simulink model "rfdc"  (R2021a)
(part 2 of 3)

      mask DialogControl t226_ADCPair23 Prompt: ADC Pair 2,3
      mask DialogControl t226_QT_adc2 Prompt: ADC 2
      mask DialogControl t226_QT_adc2_DataSettings Prompt: Data Settings
      mask DialogControl t226_QT_adc2_req_axis_clk_label Prompt: Required AXI4-Stream clock:
      mask DialogControl t226_QT_adc2_MixerSettings Prompt: MIxer Settings
      mask DialogControl t226_QT_adc2_AnalogSettings Prompt: Analog Settings
      mask DialogControl t226_QT_adc3 Prompt: ADC 3
      mask DialogControl t226_QT_adc3_DataSettings Prompt: Data Settings
      mask DialogControl t226_QT_adc3_req_axis_clk_label Prompt: Required AXI4-Stream clock:
      mask DialogControl t226_QT_adc3_MixerSettings Prompt: MIxer Settings
      mask DialogControl t226_QT_adc3_AnalogSettings Prompt: Analog Settings
      mask DialogControl t226_DualTileConfig Prompt: Dual Tile Configuration
      mask DialogControl t226_DT_adc0 Prompt: ADC 0
      mask DialogControl t226_DT_adc0_DataSettings Prompt: Data Settings
      mask DialogControl t226_DT_adc0_req_axis_clk_label Prompt: Required AXI4-Stream clock:
      mask DialogControl t226_DT_adc0_MixerSettings Prompt: MIxer Settings
      mask DialogControl t226_DT_adc0_AnalogSettings Prompt: Analog Settings
      mask DialogControl t226_DT_adc1 Prompt: ADC 1
      mask DialogControl t226_DT_adc1_DataSettings Prompt: Data Settings
      mask DialogControl t226_DT_adc1_req_axis_clk_label Prompt: Required AXI4-Stream clock:
      mask DialogControl t226_DT_adc1_MixerSettings Prompt: MIxer Settings
      mask DialogControl t226_DT_adc1_AnalogSettings Prompt: Analog Settings
      mask DialogControl Tile227_container Prompt: Tile 227
      mask DialogControl pll_clocking_config_227 Prompt: Clocking and PLL Configuration
      mask DialogControl t227_QuadTileConfig Prompt: Quad Tile Configuration
      mask DialogControl t227_ADCPair01 Prompt: ADC Pair 0,1
      mask DialogControl t227_QT_adc0 Prompt: ADC 0
      mask DialogControl t227_QT_adc0_DataSettings Prompt: Data Settings
      mask DialogControl t227_QT_adc0_req_axis_clk_label Prompt: Required AXI4-Stream clock:
      mask DialogControl t227_QT_adc0_MixerSettings Prompt: MIxer Settings
      mask DialogControl t227_QT_adc0_AnalogSettings Prompt: Analog Settings
      mask DialogControl t227_QT_adc1 Prompt: ADC 1
      mask DialogControl t227_QT_adc1_DataSettings Prompt: Data Settings
      mask DialogControl t227_QT_adc1_req_axis_clk_label Prompt: Required AXI4-Stream clock:
      mask DialogControl t227_QT_adc1_MixerSettings Prompt: MIxer Settings
      mask DialogControl t227_QT_adc1_AnalogSettings Prompt: Analog Settings
      mask DialogControl t227_ADCPair23 Prompt: ADC Pair 2,3
      mask DialogControl t227_QT_adc2 Prompt: ADC 2
      mask DialogControl t227_QT_adc2_DataSettings Prompt: Data Settings
      mask DialogControl t227_QT_adc2_req_axis_clk_label Prompt: Required AXI4-Stream clock:
      mask DialogControl t227_QT_adc2_MixerSettings Prompt: MIxer Settings
      mask DialogControl t227_QT_adc2_AnalogSettings Prompt: Analog Settings
      mask DialogControl t227_QT_adc3 Prompt: ADC 3
      mask DialogControl t227_QT_adc3_DataSettings Prompt: Data Settings
      mask DialogControl t227_QT_adc3_req_axis_clk_label Prompt: Required AXI4-Stream clock:
      mask DialogControl t227_QT_adc3_MixerSettings Prompt: MIxer Settings
      mask DialogControl t227_QT_adc3_AnalogSettings Prompt: Analog Settings
      mask DialogControl t227_DualTileConfig Prompt: Dual Tile Configuration
      mask DialogControl t227_DT_adc0 Prompt: ADC 0
      mask DialogControl t227_DT_adc0_DataSettings Prompt: Data Settings
      mask DialogControl t227_DT_adc0_req_axis_clk_label Prompt: Required AXI4-Stream clock:
      mask DialogControl t227_DT_adc0_MixerSettings Prompt: MIxer Settings
      mask DialogControl t227_DT_adc0_AnalogSettings Prompt: Analog Settings
      mask DialogControl t227_DT_adc1 Prompt: ADC 1
      mask DialogControl t227_DT_adc1_DataSettings Prompt: Data Settings
      mask DialogControl t227_DT_adc1_req_axis_clk_label Prompt: Required AXI4-Stream clock:
      mask DialogControl t227_DT_adc1_MixerSettings Prompt: MIxer Settings
      mask DialogControl t227_DT_adc1_AnalogSettings Prompt: Analog Settings
      mask DialogControl DACTileSelect Prompt: DAC Tiles
      mask DialogControl Tile228_container Prompt: Tile 228
      mask DialogControl pll_clocking_config_228 Prompt: Clocking and PLL Configuration
      mask DialogControl t228_QuadTileConfig Prompt: Quad Tile Configuration
      mask DialogControl t228_DACPair01 Prompt: DAC Pair 0,1
      mask DialogControl t228_QT_dac0 Prompt: DAC 0
      mask DialogControl t228_QT_dac0_DataSettings Prompt: Data Settings
      mask DialogControl t228_QT_dac0_req_axis_clk_label Prompt: Required AXI4-Stream clock:
      mask DialogControl t228_QT_dac0_MixerSettings Prompt: MIxer Settings
      mask DialogControl t228_QT_dac0_AnalogSettings Prompt: Analog Settings
      mask DialogControl t228_QT_dac1 Prompt: DAC 1
      mask DialogControl t228_QT_dac1_DataSettings Prompt: Data Settings
      mask DialogControl t228_QT_dac1_req_axis_clk_label Prompt: Required AXI4-Stream clock:
      mask DialogControl t228_QT_dac1_MixerSettings Prompt: MIxer Settings
      mask DialogControl t228_QT_dac1_AnalogSettings Prompt: Analog Settings
      mask DialogControl t228_DACPair23 Prompt: DAC Pair 2,3
      mask DialogControl t228_QT_dac2 Prompt: DAC 2
      mask DialogControl t228_QT_dac2_DataSettings Prompt: Data Settings
      mask DialogControl t228_QT_dac2_req_axis_clk_label Prompt: Required AXI4-Stream clock:
      mask DialogControl t228_QT_dac2_MixerSettings Prompt: MIxer Settings
      mask DialogControl t228_QT_dac2_AnalogSettings Prompt: Analog Settings
      mask DialogControl t228_QT_dac3 Prompt: DAC 3
      mask DialogControl t228_QT_dac3_DataSettings Prompt: Data Settings
      mask DialogControl t228_QT_dac3_req_axis_clk_label Prompt: Required AXI4-Stream clock:
      mask DialogControl t228_QT_dac3_MixerSettings Prompt: MIxer Settings
      mask DialogControl t228_QT_dac3_AnalogSettings Prompt: Analog Settings
      mask DialogControl t228_DualTileConfig Prompt: Dual Tile Configuration
      mask DialogControl t228_DT_dac0 Prompt: DAC 0
      mask DialogControl t228_DT_dac0_DataSettings Prompt: Data Settings
      mask DialogControl t228_DT_dac0_req_axis_clk_label Prompt: Required AXI4-Stream clock:
      mask DialogControl t228_DT_dac0_MixerSettings Prompt: MIxer Settings
      mask DialogControl t228_DT_dac0_AnalogSettings Prompt: Analog Settings
      mask DialogControl t228_DT_dac1 Prompt: DAC 1
      mask DialogControl t228_DT_dac1_DataSettings Prompt: Data Settings
      mask DialogControl t228_DT_dac1_req_axis_clk_label Prompt: Required AXI4-Stream clock:
      mask DialogControl t228_DT_dac1_MixerSettings Prompt: MIxer Settings
      mask DialogControl t228_DT_dac1_AnalogSettings Prompt: Analog Settings
      mask DialogControl Tile229_container Prompt: Tile 229
      mask DialogControl pll_clocking_config_229 Prompt: Clocking and PLL Configuration
      mask DialogControl t229_QuadTileConfig Prompt: Quad Tile Configuration
      mask DialogControl t229_DACPair01 Prompt: DAC Pair 0,1
      mask DialogControl t229_QT_dac0 Prompt: DAC 0
      mask DialogControl t229_QT_dac0_DataSettings Prompt: Data Settings
      mask DialogControl t229_QT_dac0_req_axis_clk_label Prompt: Required AXI4-Stream clock:
      mask DialogControl t229_QT_dac0_MixerSettings Prompt: MIxer Settings
      mask DialogControl t229_QT_dac0_AnalogSettings Prompt: Analog Settings
      mask DialogControl t229_QT_dac1 Prompt: DAC 1
      mask DialogControl t229_QT_dac1_DataSettings Prompt: Data Settings
      mask DialogControl t229_QT_dac1_req_axis_clk_label Prompt: Required AXI4-Stream clock:
      mask DialogControl t229_QT_dac1_MixerSettings Prompt: MIxer Settings
      mask DialogControl t229_QT_dac1_AnalogSettings Prompt: Analog Settings
      mask DialogControl t229_DACPair23 Prompt: DAC Pair 2,3
      mask DialogControl t229_QT_dac2 Prompt: DAC 2
      mask DialogControl t229_QT_dac2_DataSettings Prompt: Data Settings
      mask DialogControl t229_QT_dac2_req_axis_clk_label Prompt: Required AXI4-Stream clock:
      mask DialogControl t229_QT_dac2_MixerSettings Prompt: MIxer Settings
      mask DialogControl t229_QT_dac2_AnalogSettings Prompt: Analog Settings
      mask DialogControl t229_QT_dac3 Prompt: DAC 3
      mask DialogControl t229_QT_dac3_DataSettings Prompt: Data Settings
      mask DialogControl t229_QT_dac3_req_axis_clk_label Prompt: Required AXI4-Stream clock:
      mask DialogControl t229_QT_dac3_MixerSettings Prompt: MIxer Settings
      mask DialogControl t229_QT_dac3_AnalogSettings Prompt: Analog Settings
      mask DialogControl t229_DualTileConfig Prompt: Dual Tile Configuration
      mask DialogControl t229_DT_dac0 Prompt: DAC 0
      mask DialogControl t229_DT_dac0_DataSettings Prompt: Data Settings
      mask DialogControl t229_DT_dac0_req_axis_clk_label Prompt: Required AXI4-Stream clock:
      mask DialogControl t229_DT_dac0_MixerSettings Prompt: MIxer Settings
      mask DialogControl t229_DT_dac0_AnalogSettings Prompt: Analog Settings
      mask DialogControl t229_DT_dac1 Prompt: DAC 1
      mask DialogControl t229_DT_dac1_DataSettings Prompt: Data Settings
      mask DialogControl t229_DT_dac1_req_axis_clk_label Prompt: Required AXI4-Stream clock:
      mask DialogControl t229_DT_dac1_MixerSettings Prompt: MIxer Settings
      mask DialogControl t229_DT_dac1_AnalogSettings Prompt: Analog Settings
      mask DialogControl Tile230_container Prompt: Tile 230
      mask DialogControl pll_clocking_config_230 Prompt: Clocking and PLL Configuration
      mask DialogControl t230_QuadTileConfig Prompt: Quad Tile Configuration
      mask DialogControl t230_DACPair01 Prompt: DAC Pair 0,1
      mask DialogControl t230_QT_dac0 Prompt: DAC 0
      mask DialogControl t230_QT_dac0_DataSettings Prompt: Data Settings
      mask DialogControl t230_QT_dac0_req_axis_clk_label Prompt: Required AXI4-Stream clock:
      mask DialogControl t230_QT_dac0_MixerSettings Prompt: MIxer Settings
      mask DialogControl t230_QT_dac0_AnalogSettings Prompt: Analog Settings
      mask DialogControl t230_QT_dac1 Prompt: DAC 1
      mask DialogControl t230_QT_dac1_DataSettings Prompt: Data Settings
      mask DialogControl t230_QT_dac1_req_axis_clk_label Prompt: Required AXI4-Stream clock:
      mask DialogControl t230_QT_dac1_MixerSettings Prompt: MIxer Settings
      mask DialogControl t230_QT_dac1_AnalogSettings Prompt: Analog Settings
      mask DialogControl t230_DACPair23 Prompt: DAC Pair 2,3
      mask DialogControl t230_QT_dac2 Prompt: DAC 2
      mask DialogControl t230_QT_dac2_DataSettings Prompt: Data Settings
      mask DialogControl t230_QT_dac2_req_axis_clk_label Prompt: Required AXI4-Stream clock:
      mask DialogControl t230_QT_dac2_MixerSettings Prompt: MIxer Settings
      mask DialogControl t230_QT_dac2_AnalogSettings Prompt: Analog Settings
      mask DialogControl t230_QT_dac3 Prompt: DAC 3
      mask DialogControl t230_QT_dac3_DataSettings Prompt: Data Settings
      mask DialogControl t230_QT_dac3_req_axis_clk_label Prompt: Required AXI4-Stream clock:
      mask DialogControl t230_QT_dac3_MixerSettings Prompt: MIxer Settings
      mask DialogControl t230_QT_dac3_AnalogSettings Prompt: Analog Settings
      mask DialogControl t230_DualTileConfig Prompt: Dual Tile Configuration
      mask DialogControl t230_DT_dac0 Prompt: DAC 0
      mask DialogControl t230_DT_dac0_DataSettings Prompt: Data Settings
      mask DialogControl t230_DT_dac0_req_axis_clk_label Prompt: Required AXI4-Stream clock:
      mask DialogControl t230_DT_dac0_MixerSettings Prompt: MIxer Settings
      mask DialogControl t230_DT_dac0_AnalogSettings Prompt: Analog Settings
      mask DialogControl t230_DT_dac1 Prompt: DAC 1
      mask DialogControl t230_DT_dac1_DataSettings Prompt: Data Settings
      mask DialogControl t230_DT_dac1_req_axis_clk_label Prompt: Required AXI4-Stream clock:
      mask DialogControl t230_DT_dac1_MixerSettings Prompt: MIxer Settings
      mask DialogControl t230_DT_dac1_AnalogSettings Prompt: Analog Settings
      mask DialogControl Tile231_container Prompt: Tile 231
      mask DialogControl pll_clocking_config_231 Prompt: Clocking and PLL Configuration
      mask DialogControl t231_QuadTileConfig Prompt: Quad Tile Configuration
      mask DialogControl t231_DACPair01 Prompt: DAC Pair 0,1
      mask DialogControl t231_QT_dac0 Prompt: DAC 0
      mask DialogControl t231_QT_dac0_DataSettings Prompt: Data Settings
      mask DialogControl t231_QT_dac0_req_axis_clk_label Prompt: Required AXI4-Stream clock:
      mask DialogControl t231_QT_dac0_MixerSettings Prompt: MIxer Settings
      mask DialogControl t231_QT_dac0_AnalogSettings Prompt: Analog Settings
      mask DialogControl t231_QT_dac1 Prompt: DAC 1
      mask DialogControl t231_QT_dac1_DataSettings Prompt: Data Settings
      mask DialogControl t231_QT_dac1_req_axis_clk_label Prompt: Required AXI4-Stream clock:
      mask DialogControl t231_QT_dac1_MixerSettings Prompt: MIxer Settings
      mask DialogControl t231_QT_dac1_AnalogSettings Prompt: Analog Settings
      mask DialogControl t231_DACPair23 Prompt: DAC Pair 2,3
      mask DialogControl t231_QT_dac2 Prompt: DAC 2
      mask DialogControl t231_QT_dac2_DataSettings Prompt: Data Settings
      mask DialogControl t231_QT_dac2_req_axis_clk_label Prompt: Required AXI4-Stream clock:
      mask DialogControl t231_QT_dac2_MixerSettings Prompt: MIxer Settings
      mask DialogControl t231_QT_dac2_AnalogSettings Prompt: Analog Settings
      mask DialogControl t231_QT_dac3 Prompt: DAC 3
      mask DialogControl t231_QT_dac3_DataSettings Prompt: Data Settings
      mask DialogControl t231_QT_dac3_req_axis_clk_label Prompt: Required AXI4-Stream clock:
      mask DialogControl t231_QT_dac3_MixerSettings Prompt: MIxer Settings
      mask DialogControl t231_QT_dac3_AnalogSettings Prompt: Analog Settings
      mask DialogControl t231_DualTileConfig Prompt: Dual Tile Configuration
      mask DialogControl t231_DT_dac0 Prompt: DAC 0
      mask DialogControl t231_DT_dac0_DataSettings Prompt: Data Settings
      mask DialogControl t231_DT_dac0_req_axis_clk_label Prompt: Required AXI4-Stream clock:
      mask DialogControl t231_DT_dac0_MixerSettings Prompt: MIxer Settings
      mask DialogControl t231_DT_dac0_AnalogSettings Prompt: Analog Settings
      mask DialogControl t231_DT_dac1 Prompt: DAC 1
      mask DialogControl t231_DT_dac1_DataSettings Prompt: Data Settings
      mask DialogControl t231_DT_dac1_req_axis_clk_label Prompt: Required AXI4-Stream clock:
      mask DialogControl t231_DT_dac1_MixerSettings Prompt: MIxer Settings
      mask DialogControl t231_DT_dac1_AnalogSettings Prompt: Analog Settings
      mask DialogControl SystemClocking Prompt: System Clocking And Real-time Ports
      mask DialogControl ADCClocking Prompt: ADC Tile Clocking
      mask DialogControl t224_clock_config Prompt: ADC Tile 224
      mask DialogControl t225_clock_config Prompt: ADC Tile 225
      mask DialogControl t226_clock_config Prompt: ADC Tile 226
      mask DialogControl t227_clock_config Prompt: ADC Tile 227
      mask DialogControl DACClocking Prompt: DAC Tile Clocking
      mask DialogControl t228_clock_config Prompt: DAC Tile 228
      mask DialogControl t229_clock_config Prompt: DAC Tile 229
      mask DialogControl t230_clock_config Prompt: DAC Tile 230
      mask DialogControl t231_clock_config Prompt: DAC Tile 231
